simulink model "pm"  (R2023b)
settings: Solver=VariableStepAuto  StartTime=0.0  StopTime=100  MaxStep=0.0001  RelTol=1e-8
settings Model: Creator=Хз_переименуюсь  LastModifiedBy=Хз_переименуюсь

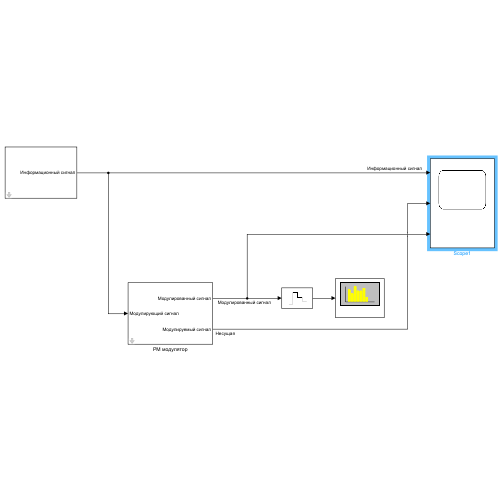
[thumbnail: Simulink's stored preview of the top-level diagram]
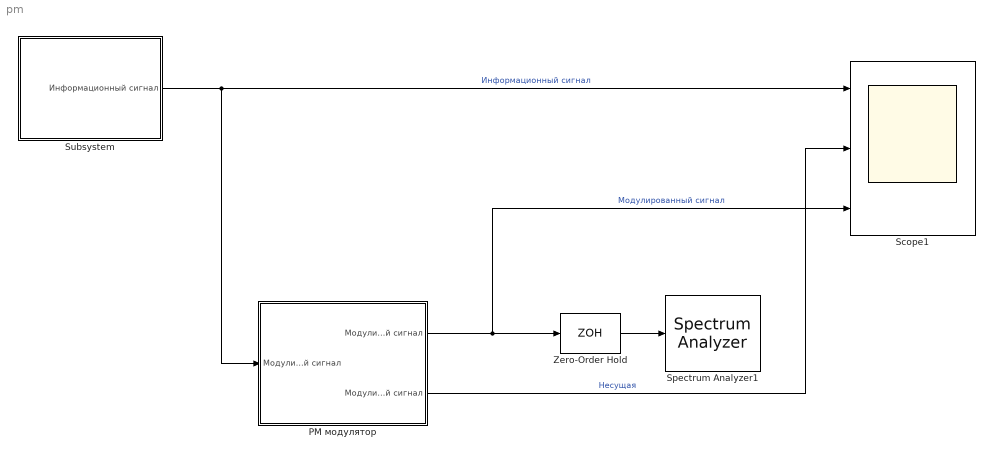
== system pm ==
  PM модулятор : Subsystem  mask{Fc=1000, Dphi=2*pi}
      mask prompts: Fc "Частота несущей, Гц"; Dphi "Девиация Фазы"
  Scope1 : Scope  NumInputPorts=3
  Spectrum Analyzer1 : SpectrumAnalyzer  WindowPosition=[1.000000,41.000000,1539.000000,940.000000,]  ScopeFrameLocation=window  FrequencySpan=Start and stop frequencies  Span=1000  StartFrequency=0  StopFrequency=500  YLimits=[-155.83550136,-15.53135504]
      settings: OpenAtSimulationStart=off
  Subsystem : Subsystem  mask{F1=0, F2=0, F3=0, F4=100}
      mask prompts: F1 "Частота1, Гц"; F2 "Частота1, Гц"; F3 "Частота3, Гц"; F4 "Частота4, Гц"
      mask DialogControl asdfsfdg Prompt: Parameters
  Zero-Order Hold : ZeroOrderHold  SampleTime=1e-3
  wires:
  Zero-Order Hold/1 -> Spectrum Analyzer1/1
  Subsystem/1(Информационный сигнал) -> PM модулятор/1(Модулирующий сигнал), Scope1/1  "Информационный сигнал"
  PM модулятор/2(Модулируемый сигнал) -> Scope1/2  "Несущая"
  PM модулятор/1(Модулированный сигнал) -> Zero-Order Hold/1, Scope1/3  "Модулированный сигнал"

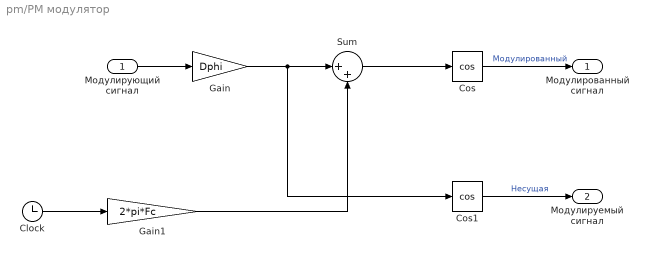
== system pm/PM модулятор ==
  Модулирующий сигнал : Inport
  Clock : Clock
  Cos : Trigonometry  Operator=cos
  Cos1 : Trigonometry  Operator=cos
  Gain : Gain  Gain=Dphi
  Gain1 : Gain  Gain=2*pi*Fc
  Sum : Sum  Inputs=|++
  Модулированный сигнал : Outport
  Модулируемый сигнал : Outport  Port=2
  wires:
  Модулирующий сигнал/1 -> Gain/1
  Sum/1 -> Cos/1
  Gain/1 -> Cos1/1, Sum/1
  Cos/1 -> Модулированный сигнал/1  "Модулированный"
  Cos1/1 -> Модулируемый сигнал/1  "Несущая"
  Clock/1 -> Gain1/1
  Gain1/1 -> Sum/2

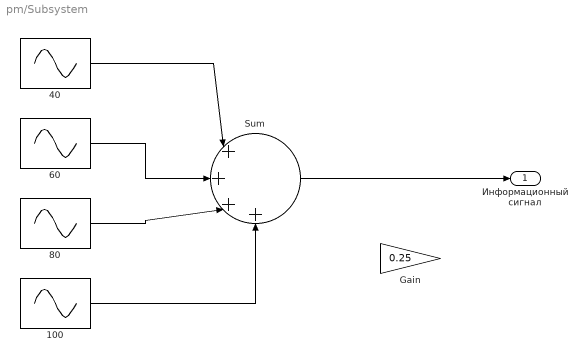
== system pm/Subsystem ==
  100 : Sin  Frequency=2*pi*F4  SampleTime=0
  40 : Sin  Frequency=2*pi*F1  SampleTime=0
  60 : Sin  Frequency=2*pi*F2  SampleTime=0
  80 : Sin  Frequency=2*pi*F3  SampleTime=0
  Gain : Gain  Gain=0.25
  Sum : Sum  Inputs=|++++
  Информационный сигнал : Outport
  wires:
  40/1 -> Sum/1
  60/1 -> Sum/2
  80/1 -> Sum/3
  100/1 -> Sum/4
  Sum/1 -> Информационный сигнал/1
